simulink model "MIMO_BPSK_Alamouti_RTLRx"  (R2026a)
settings: Solver=FixedStepDiscrete  StopTime=5
PreLoadFcn:
  | PayloadBitRate = 250e3/4
  | 
  | EbNo = 15;
  | 
  | barker=[+1 +1 +1 +1 +1 -1 -1 +1 +1 -1 +1 -1 +1].' > 0;
  | hModulator = comm.BPSKModulator;
  | hModulator.PhaseOffset = 0;
  | modHeader = step(hModulator, barker);
model workspace: external: MAT-File modelspace.mat (data not in the file)
undefined symbols (not defined in the file or in its folder): gcbh, rcfiltgaincompat
libraries: commrfcorlib x2, commsync2 x2, sdrrlib x1, commrflib2 x1, commmimo x1, commdigbbndpm3 x1, commfilt2 x1
settings Model: LastModifiedBy=dawn
settings DataIOCC: SignalLoggingSaveFormat=ModelDataLogs
settings DebuggingCC: UnderspecifiedInitializationDetection=Classic
settings HardwareCC: ProdHWDeviceType=32-bit Generic
settings GRTTargetCC: CombineOutputUpdateFcns=off  GRTInterface=on

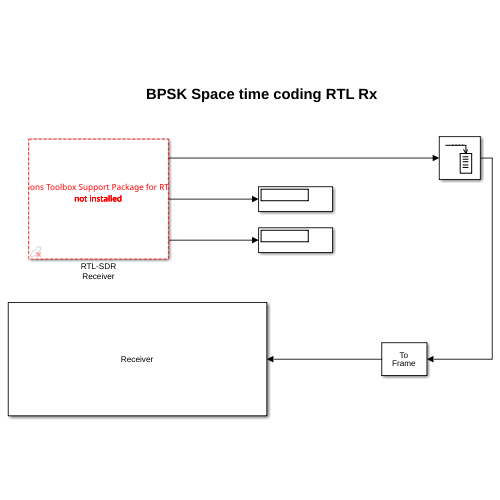
[thumbnail: Simulink's stored preview of the top-level diagram]
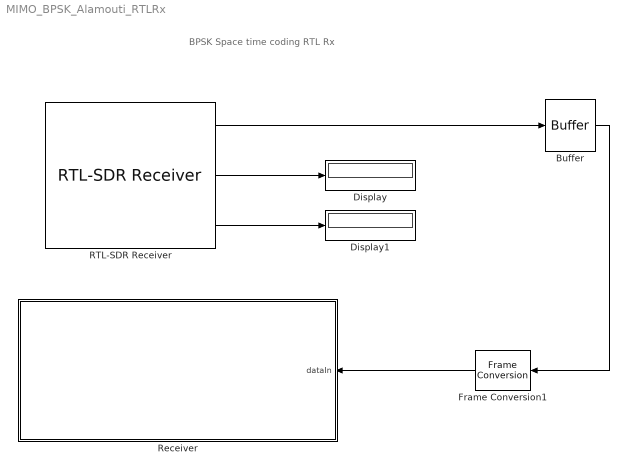
== system MIMO_BPSK_Alamouti_RTLRx ==
  note: BPSK Space time coding RTL Rx
  Buffer : Buffer  N=2324  OutputFrames=off
  Display : Display
  Display1 : Display
  Frame Conversion1 : FrameConversion
  RTL-SDR Receiver : sdrrlib/RTL-SDR Receiver  IPAddress=0  CenterFrequencySource=Dialog  CenterFrequency=921e6  GainSource=Dialog  Gain=10  ADCRate=250e3  FrequencyCorrection=1  LostSamplesOutputPort=on  LatencyOutputPort=on  OutputDataType=double  FrameLength=4096*16  EnableBurstMode=off  NumFramesInBurst=20  sobjType=sdrr.internal.SDRRTLReceiverSL  dataUDPPort=-1  ctrlUDPPort=-1  subDeviceList=nosubdev  sdrBlockType=SDRBlockTypeSLT.SDRRxBlock  requester=UNUSED_BY_SFCN  sdrExecutionMode=SDRExecutionModeSLT.ExecModeHW  BypassUserLogic=off  DecimatorSelect=DDC decimator  SourceSelect=RF data  SineAmplitude=16000  EnableInternalClock=off  BypassIQBalance=off  IFBandwidth=40e6  ADCRateSource=Dialog  IntermediateFrequency=0  DecimationFactorSource=Dialog  DecimationFactor=512  RFFrequencyIsTunable=logical(0)  SampleTime=(4096*16)/(250e3)  IFBandwidthSource=Dialog  SineFrequency=30000  BypassDCBlockingFilter=off  IntermediateFrequencySource=Dialog  IQBalanceCoefficients=64  SkipAllHardwareResetAndInitialization=off  EnableIQCalibrationTable=on  CacheIQCalibrationTable=off  EnableOffsetTuning=off  EnableRTLAGC=off  EnableTestMode=off  EnableTunerAGC=off  FrequencyCorrectionSource=Dialog  NumMLBuffers=128  NumUSBBuffers=16  RTLCrystalFrequency=28800000  TunerCrystalFrequency=28800000
  Receiver : Subsystem
      mask Display: disp('Receiver')
  wires:
  Frame Conversion1/1 -> Receiver/1(dataIn)
  RTL-SDR Receiver/1 -> Buffer/1
  Buffer/1 -> Frame Conversion1/1
  RTL-SDR Receiver/2 -> Display/1
  RTL-SDR Receiver/3 -> Display1/1

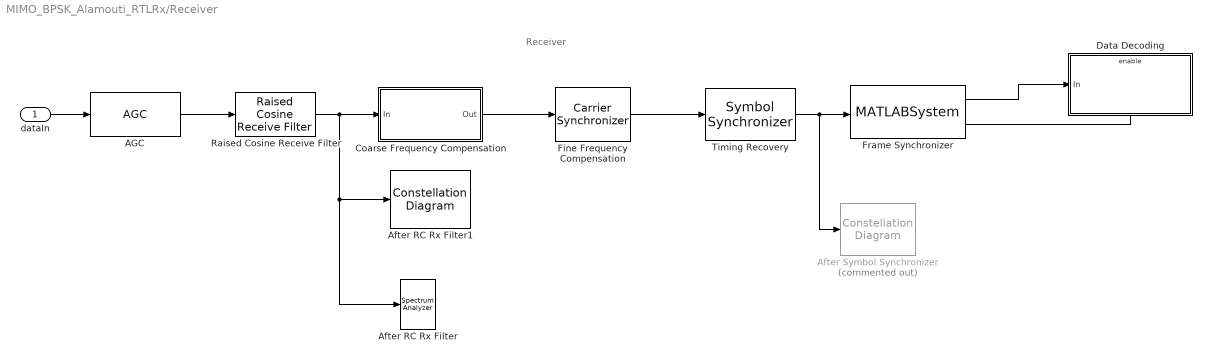
== system MIMO_BPSK_Alamouti_RTLRx/Receiver ==
  note: Receiver
  dataIn : Inport
  AGC : commrfcorlib/AGC  LegacyMode=off  DetectorMethod=Rectifier  LoopMethod=Linear  UpdatePeriod=100  StepSize=0.1  AdaptationStepSize=0.01  DesiredOutputPower=1/sqrt(4)/2  AveragingLength=2324  MaximumGain=30  MaxPowerGain=50  GainOutputPort=off  InputPowerOutputPort=off  SimulateUsing=Code generation
  After RC Rx Filter : SpectrumAnalyzer  WindowPosition=[550.000000,321.000000,800.000000,500.000000,]  ScopeFrameLocation=window  Method=Welch  SampleRate=129687.5  RBWSource=Property  RBW=75  FFTLength=128  Span=100000  StartFrequency=-50000  StopFrequency=50000  AveragingMethod=Running  SpectralAverages=2  SpectrumUnits=dBW  Title=After Raised Cosine Rx Filter  YLabel=Power Spectrum  YLimits=[-138.6333 1.2252]  ShowGrid=off  AllowFFTLengthLessThanSamplesPerUpdate=on  DefaultConfigurationName=spbscopes.SpectrumAnalyzerBlockCfg  IsFrequencyInputMode=0  FrequencyVectorPort=0  FrequencyVectorFromPort=0  FrequencyInputRBWPort=0  FrequencyInputRBWFromPort=0
  After RC Rx Filter1 : ConstellationDiagram  Tag=ScatterPlot  WindowPosition=[818.000000,532.000000,401.000000,517.000000,]  ScopeFrameLocation=window  SamplesPerSymbol=2  SymbolsToDisplaySource=Property  SymbolsToDisplay=1000  ReferenceConstellation=BPSK  Title=After Raised Cosine Rx Filter  XLimits=[-1.25 1.25]  YLimits=[-1.25 1.25]  AxesLimits=[-1.25 1.25]  DefaultConfigurationName=comm.scopes.ConstellationDiagramBlockCfg
  After Symbol Synchronizer : ConstellationDiagram  Tag=ScatterPlot  Commented=on  WindowPosition=[1436.000000,665.000000,403.000000,337.000000,]  ScopeFrameLocation=window  SamplesPerSymbol=2  SymbolsToDisplaySource=Property  SymbolsToDisplay=1000  ReferenceConstellation=BPSK  Title=After Symbol Synchronizer  XLimits=[-1.25 1.25]  YLimits=[-1.25 1.25]  AxesLimits=[-1.25 1.25]  DefaultConfigurationName=comm.scopes.ConstellationDiagramBlockCfg
  Coarse Frequency Compensation : Subsystem
      mask Display: disp('Coarse Frequency\nCompensation');
  Data Decoding : Subsystem
      mask Display: disp('Data Decoding');
  Fine Frequency Compensation : commsync2/Carrier Synchronizer  Modulation=BPSK  ModulationPhaseOffset=Custom  CustomPhaseOffset=0  SamplesPerSymbol=2  DampingFactor=1  NormalizedLoopBandwidth=0.01  EstimatedPhaseErrorOutputPort=off  SimulateUsing=Code generation
  Frame Synchronizer : MATLABSystem  System=FrameFormation  OutputFrameLength=581  PerformSynchronization=on  InternalBufferLength=300  FrameHeader=modHeader  SimulateUsing=Interpreted execution
  Raised Cosine Receive Filter : commfilt2/Raised Cosine Receive Filter  filtType=Square root  R=0.5  filtSpan=10  N=4  downFactor=2  downOffset=0  filterGain=rcfiltgaincompat(gcbh)  InputProcessing=Columns as channels (frame based)  RateOptions=Enforce single-rate processing  framing=Enforce single-rate processing  checkCoeff=off  variableName=rcRxFilt1  currentFiltSpan=10  D=(10)/2  inputOffset=0  sampMode=Mute  saveAsFlag=0  rateMode=Downsampling  checkGain=Normalized  launchFVT=off  roundingMode=Floor  overflowMode=off  coeffDataTypeStr=Inherit: Same word length as input  coeffMin=[]  coeffMax=[]  coeffLastDataTypeStr=Inherit: Same word length as input  accumDataTypeStr=Inherit: Same as product output  accumLastDataTypeStr=Inherit: Same as product output  outputDataTypeStr=Inherit: Same as accumulator  outputMin=[]  outputMax=[]  outputLastDataTypeStr=Inherit: Same as accumulator
  Timing Recovery : commsync2/Symbol Synchronizer  Modulation=PAM/PSK/QAM  TimingErrorDetector=Early-Late (non-data-aided)  SamplesPerSymbol=2  DampingFactor=1  NormalizedLoopBandwidth=0.01  DetectorGain=5.4  TimingErrorOutputPort=off  SimulateUsing=Code generation
  wires:
  Frame Synchronizer/1 -> Data Decoding/1(In)
  Frame Synchronizer/2 -> Data Decoding/Enable
  Raised Cosine Receive Filter/1 -> Coarse Frequency Compensation/1(In), After RC Rx Filter1/1, After RC Rx Filter/1
  Coarse Frequency Compensation/1(Out) -> Fine Frequency Compensation/1
  Fine Frequency Compensation/1 -> Timing Recovery/1
  dataIn/1 -> AGC/1
  AGC/1 -> Raised Cosine Receive Filter/1
  Timing Recovery/1 -> Frame Synchronizer/1, After Symbol Synchronizer/1

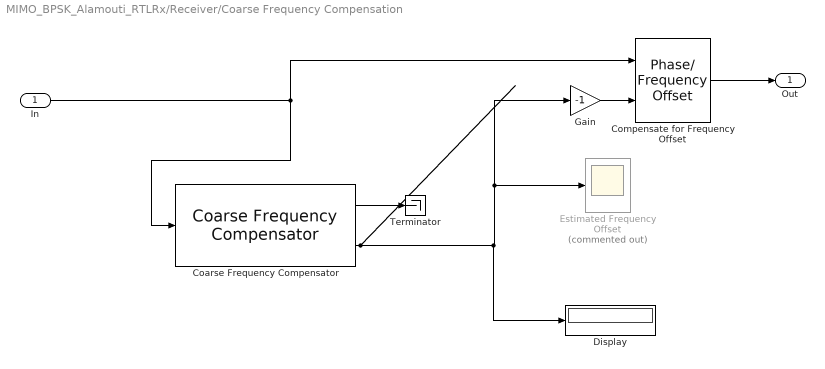
== system MIMO_BPSK_Alamouti_RTLRx/Receiver/Coarse Frequency Compensation ==
  In : Inport
  Coarse Frequency Compensator : commrfcorlib/Coarse Frequency Compensator  Modulation=BPSK  Algorithm=FFT-based  FrequencyResolution=50  MaximumFrequencyOffset=5e3  SamplesPerSymbol=4  EstimatedFreqOffsetPort=on  SimulateUsing=Code generation
  Compensate for Frequency Offset : commrflib2/Phase// Frequency Offset  PhaseOffset=0  FrequencyOffsetFromPort=on  FrequencyOffset=100  SimulateUsing=Code generation
  Display : Display
  Estimated Frequency Offset : Scope  Commented=on
      settings: TimeSpan=0.1  TimeUnits=Metric (based on Time Span)  ActiveDisplayYMinimum=4004.88  ActiveDisplayYMaximum=6004.88  YLabel=Estimated Frequency Offset (Hz)  DataLoggingVariableName=ScopeDataEFO
  Gain : Gain  Gain=-1
  Terminator : Terminator
  Out : Outport  VectorParamsAs1DForOutWhenUnconnected=off
  wires:
  In/1 -> Coarse Frequency Compensator/1, Compensate for Frequency Offset/1
  Compensate for Frequency Offset/1 -> Out/1
  Gain/1 -> Compensate for Frequency Offset/2
  Coarse Frequency Compensator/1 -> Terminator/1
  Coarse Frequency Compensator/2 -> Display/1, Estimated Frequency Offset/1, Gain/1

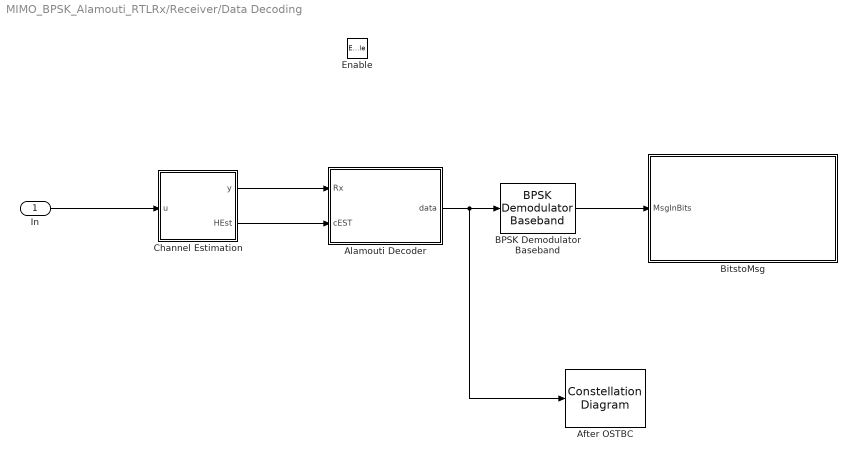
== system MIMO_BPSK_Alamouti_RTLRx/Receiver/Data Decoding ==
  In : Inport
  Enable : EnablePort
  After OSTBC : ConstellationDiagram  Tag=ScatterPlot  WindowPosition=[1488.000000,170.000000,285.000000,338.000000,]  ScopeFrameLocation=window  SamplesPerSymbol=2  SymbolsToDisplaySource=Property  SymbolsToDisplay=1000  ReferenceConstellation=BPSK  Title=After Space time coding  XLimits=[-2.876 2.8997]  YLimits=[-2.876 2.8997]  AxesLimits=[-2.876 2.8997]  ShowLegend=on  DefaultConfigurationName=comm.scopes.ConstellationDiagramBlockCfg
  Alamouti Decoder : Subsystem  mask(Constant){Select_2=2}
      mask prompts: Select_2 "Decoder Selection"
      mask help:
      | Decoder Selection Parameter
      | 1 Simulink Block
      | 2 User Defined Function
  BPSK Demodulator Baseband : commdigbbndpm3/BPSK Demodulator Baseband  DecType=Hard decision  VarSource=Dialog  Variance=1  Ph=0  outDtype=double  derotateFactorWordLen=16  derotateFactorDataTypeStr=Inherit: Same word length as input  derotateFactorLastDataTypeStr=Inherit: Same word length as input
  BitstoMsg : MATLAB Function  TreatAsAtomicUnit=on
  Channel Estimation : MATLAB Function  TreatAsAtomicUnit=on
  wires:
  In/1 -> Channel Estimation/1(u)
  Alamouti Decoder/1(data) -> After OSTBC/1, BPSK Demodulator Baseband/1
  Channel Estimation/1(y) -> Alamouti Decoder/1(Rx)
  Channel Estimation/2(HEst) -> Alamouti Decoder/2(cEST)
  BPSK Demodulator Baseband/1 -> BitstoMsg/1(MsgInBits)

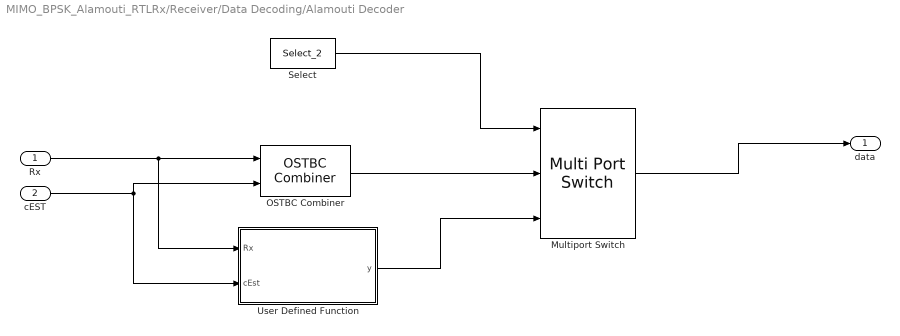
== system MIMO_BPSK_Alamouti_RTLRx/Receiver/Data Decoding/Alamouti Decoder ==
  Rx : Inport
  cEST : Inport  Port=2
  Multiport Switch : MultiPortSwitch  Inputs=2  SaturateOnIntegerOverflow=off  InputSameDT=off
  OSTBC Combiner : commmimo/OSTBC Combiner  numTx=2  rate=3/4  numRx=1  roundingMode=Floor  overflowMode=Wrap  OvFlMode=off  OvFlModeLastStrValue=off  crossProductWordLen=32  crossProductFracLen=16  crossSumWordLen=32  crossSumFracLen=16  egyProductWordLen=32  egyProductFracLen=16  egySumWordLen=32  egySumFracLen=16  divisionWordLen=32  divisionFracLen=16  divisionDataTypeStr=Inherit: Same as accumulator  divisionLastDataTypeStr=Inherit: Same as accumulator
  Select : Constant  Value=Select_2  VectorParams1D=off  OutMin=1  OutMax=5  OutDataTypeStr=Inherit: Inherit via back propagation
  "User Defined Function " : MATLAB Function  TreatAsAtomicUnit=on
  data : Outport  VectorParamsAs1DForOutWhenUnconnected=off
  wires:
  Select/1 -> Multiport Switch/1
  Rx/1 -> OSTBC Combiner/1, "User Defined Function "/1(Rx)
  cEST/1 -> OSTBC Combiner/2, "User Defined Function "/2(cEst)
  OSTBC Combiner/1 -> Multiport Switch/2
  "User Defined Function "/1(y) -> Multiport Switch/3
  Multiport Switch/1 -> data/1

== matlab function MIMO_BPSK_Alamouti_RTLRx/Receiver/Data Decoding/Channel Estimation ==
  data: u input; y output size=[560, 1]; HEst output
function [y, HEst] = fcn(u)
%incomplete code
HEst = complex(zeros(560, 2));
y=u(22:581);

== matlab function MIMO_BPSK_Alamouti_RTLRx/Receiver/Data Decoding/Alamouti Decoder/User Defined Function  ==
  data: Rx input; y output size=[560, 1]; cEst input
function y = Alamouti_decoder(Rx, cEst)
%incomplete code
y=complex(zeros(560,1));

== matlab function MIMO_BPSK_Alamouti_RTLRx/Receiver/Data Decoding/BitstoMsg ==
  data: MsgInBits input; NumFrameDetected data_store_memory; SystemBER data_store_memory
function BitstoMsg(MsgInBits)

% Configuration paramters
PayloadMessage = 'Welcome to the school of electrical and information engineering, Uni. of Sydney!';
NumBitsPerCharacter  = 7;
global NumFrameDetected;    %count the number of frame correctly received
global SystemBER;
coder.extrinsic('dec2bin','fprintf','num2str');
%% Alorithm

NumFrameDetected=NumFrameDetected+1;     
if NumFrameDetected>1 % Display every frame after the first.
    % transmitted message

    txMsgInBits    = coder.const(double(dec2bin(PayloadMessage, NumBitsPerCharacter).'));
    txMsgInBits    = txMsgInBits(:) - 48;
    bitMsgLen      = length(txMsgInBits);

    % received message
    %remove padding
    rxMsgInBits = MsgInBits(1:bitMsgLen,:);
    % disp(rxMsgInBits);
    decMsgInBits = reshape(rxMsgInBits(1:bitMsgLen),[7, bitMsgLen/7])';
    %decMsgInBits = reshape(rxMsgInBits(1:bitMsgLen),[bitMsgLen/7, 7]);
    disp('Received Message:');
    disp(char(bin2dec(num2str(decMsgInBits)))');

    %% BER
    % BER calculation
    numBitErr = sum(txMsgInBits(:) ~= rxMsgInBits(:));
    BER = numBitErr/(bitMsgLen);
    
    SystemBER = (SystemBER*(NumFrameDetected-1) + BER)/NumFrameDetected;%accumulated BER
    fprintf('Error Stats:\nTotal number of Frame detected = %d.  The System average BER = %f\n\n', ...
             NumFrameDetected, SystemBER);
 end
